simulink model "pid_controller"  (R2025b)
settings: Solver=VariableStepAuto  StartTime=0.0  StopTime=10  RelTol=1e-3
values from neighbouring files (symbols this model uses):
  Kd = 10.0    [pid_constants.sldd]
  Ki = 200.0    [pid_constants.sldd]
  Kp = 100.0    [pid_constants.sldd]
settings Model: DataDictionary=pid_constants.sldd  Creator=R  LastModifiedBy=R
settings ModelReferenceCC: ModelReferenceMinAlgLoopOccurrences=on

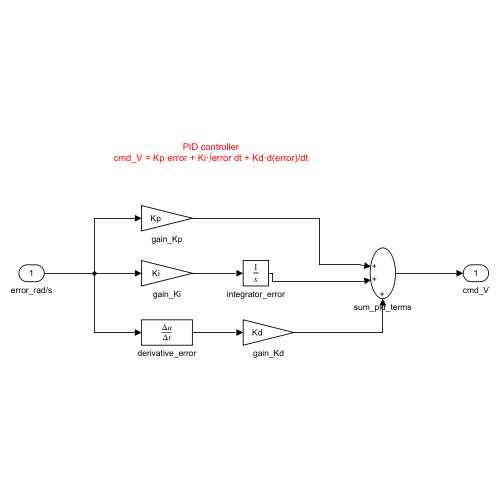
[thumbnail: Simulink's stored preview of the top-level diagram]
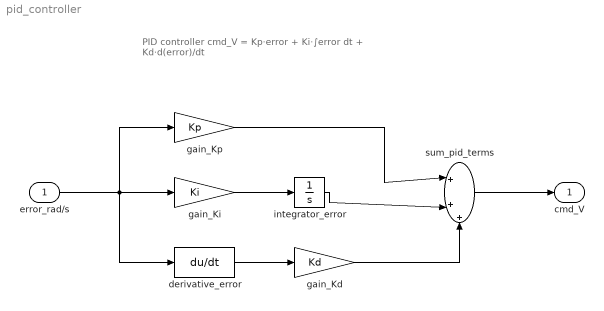
== system pid_controller ==
  note: PID controller
      | cmd_V = Kp·error + Ki·∫error dt + Kd·d(error)/dt
  error_rad/s : Inport
  derivative_error : Derivative
  gain_Kd : Gain  Gain=Kd
  gain_Ki : Gain  Gain=Ki
  gain_Kp : Gain  Gain=Kp
  integrator_error : Integrator
  sum_pid_terms : Sum  Inputs=|+++
  cmd_V : Outport
  wires:
  error_rad/s/1 -> gain_Kp/1, gain_Ki/1, derivative_error/1
  gain_Ki/1 -> integrator_error/1
  derivative_error/1 -> gain_Kd/1
  gain_Kp/1 -> sum_pid_terms/1
  integrator_error/1 -> sum_pid_terms/2
  gain_Kd/1 -> sum_pid_terms/3
  sum_pid_terms/1 -> cmd_V/1
